simulink model "turbo_controller"  (R2025a)
settings: Solver=FixedStepAuto  StartTime=0.0  StopTime=inf  FixedStep=0.001  RelTol=1e-3
PostLoadFcn:
  | % 自动定位同目录CubeMX文件；不需要外部初始化脚本。
  | codertarget.data.setParameterValue('turbo_controller','STM32CubeMX.ProjectFile',fullfile(fileparts(get_param('turbo_controller','FileName')),'turbo_f407.ioc'));
InitFcn:
  | % 中文说明：按原控制器字段与类型创建三组接口总线；控制参数已内嵌。
  | tc_names=["EValve_Cycle" "EValve_Open" "Eblast_Cycle" "Eblast_Open" "Motor_Cycle" "Motor_Open" "EValve_Enable" "Eblast_Enable" "Motor_Enable" "SWO_Firework" "SWO_BleedAir" "EngineState" "Flag_ECUReset_Clear" "Flag_ECUReset_Save" "Flag_Reset_Enable" "Accelerator" "Nc_dem" "Nc"]; tc_types=["uint16" "uint16" "uint16" "uint16" "uint16" "uint16" "uint8" "uint8" "uint8" "uint8" "uint8" "uint8" "uint8" "uint8" "uint8" "single" "single" "single"];
  | for tc_k=1:numel(tc_names)
  |  tc_e(tc_k)=Simulink.BusElement; tc_e(tc_k).Name=char(tc_names(tc_k)); tc_e(tc_k).DataType=char(tc_types(tc_k));
  | end
  | EngineControl_Out=Simulink.Bus; EngineControl_Out.DataScope='Exported'; EngineControl_Out.Elements=tc_e;
  | clear tc_e tc_names tc_types tc_k
  | tc_names=["savedata1" "savedata2" "savedata3" "savedata4" "savedata5" "savedata6" "savedata7" "savedata8" "savedata9" "savedata10" "savedata11" "savedata12" "savedata13" "savedata14" "savedata15" "savedata16" "savedata17" "savedata18" "savedata19" "savedata20" "savedata21" "savedata22" "savedata23" "savedata24" "savedata25"]; tc_types=["single" "single" "single" "single" "single" "single" "single" "single" "single" "single" "single" "single" "single" "single" "single" "single" "single" "single" "single" "single" "single" "single" "single" "single" "single"];
  | for tc_k=1:numel(tc_names)
  |  tc_e(tc_k)=Simulink.BusElement; tc_e(tc_k).Name=char(tc_names(tc_k)); tc_e(tc_k).DataType=char(tc_types(tc_k));
  | end
  | SaveData_Out=Simulink.Bus; SaveData_Out.DataScope='Exported'; SaveData_Out.Elements=tc_e;
  | clear tc_e tc_names tc_types tc_k
  | tc_names=["senddata1" "senddata2" "senddata3" "senddata4" "senddata5" "senddata6" "senddata7" "senddata8" "senddata9" "senddata10" "senddata11" "senddata12" "senddata13" "senddata14" "senddata15" "senddata16" "senddata17" "senddata18" "senddata19" "senddata20" "senddata21" "senddata22" "senddata23" "senddata24" "senddata25" "senddata26" "senddata27" "senddata28" "senddata29"]; tc_types=["uint8" "uint8" "uint8" "uint8" "uint8" "uint8" "uint8" "uint8" "uint8" "uint8" "uint8" "uint8" "uint8" "uint8" "uint8" "uint8" "uint8" "uint8" "uint8" "uint8" "uint8" "uint8" "uint8" "uint8" "uint8" "uint8" "uint8" "uint8" "uint8"];
  | for tc_k=1:numel(tc_names)
  |  tc_e(tc_k)=Simulink.BusElement; tc_e(tc_k).Name=char(tc_names(tc_k)); tc_e(tc_k).DataType=char(tc_types(tc_k));
  | end
  | SendData_Out=Simulink.Bus; SendData_Out.DataScope='Exported'; SendData_Out.Elements=tc_e;
  | clear tc_e tc_names tc_types tc_k
  | 
  | % 以下为接口中文说明；只设置描述，不改变数值或数据类型。
  | EngineControl_Out.Description='执行控制输出（阀、电机、点火、状态及复位请求）';
  | tc_cn=["EValve_Cycle（主油阀周期计数（每计数2毫秒））" "EValve_Open（主油阀开通计数（每计数2毫秒））" "Eblast_Cycle（副油阀周期计数（每计数2毫秒））" "Eblast_Open（副油阀开通计数（每计数2毫秒））" "Motor_Cycle（起动电机周期计数）" "Motor_Open（起动电机开通计数）" "EValve_Enable（主油阀驱动使能）" "Eblast_Enable（副油阀驱动使能）" "Motor_Enable（起动电机使能）" "SWO_Firework（点火器使能（1开））" "SWO_BleedAir（引气阀使能（1开））" "EngineState（发动机状态）" "Flag_ECUReset_Clear（清除复位恢复状态请求）" "Flag_ECUReset_Save（保存复位恢复数据请求）" "Flag_Reset_Enable（处理器软件复位请求）" "Accelerator（油门／油泵给定控制量）" "Nc_dem（控制目标转速）" "Nc（发动机反馈转速（转每分））"];
  | tc_elements=EngineControl_Out.Elements;
  | for tc_k=1:numel(tc_cn)
  |  tc_elements(tc_k).Description=char(tc_cn(tc_k));
  | end
  | EngineControl_Out.Elements=tc_elements;
  | clear tc_cn tc_elements tc_k
  | SaveData_Out.Description='25项运行记录；字段含义按当前模型数据来源解释';
  | tc_cn=["savedata1（指令回显记录）" "savedata2（入口总温记录（℃））" "savedata3（电源电压记录）" "savedata4（排气温度记录（℃））" "savedata5（标定燃油压力记录）" "savedata6（副油阀占空比记录（％））" "savedata7（主油阀占空比记录（％））" "savedata8（温度修正转速记录）" "savedata9（开关输出及反馈位域）" "savedata10（物理转速记录）" "savedata11（油泵目标给定原始值）" "savedata12（起动电机占空比记录（％））" "savedata13（发动机状态码记录）" "savedata14（故障告警位域记录）" "savedata15（模型记录帧序号）" "savedata16（处理器温度记录（℃））" "savedata17（装订转速记录（沿用旧电源字段名））" "savedata18（导航高度记录）" "savedata19（飞行空速记录）" "savedata20（主阀旧记录位（恒零保留））" "savedata21（第21项保留记录（恒零））" "savedata22（保留记录项22）" "savedata23（保留记录项23）" "savedata24（保留记录项24）" "savedata25（保留记录项25）"];
  | tc_elements=SaveData_Out.Elements;
  | for tc_k=1:numel(tc_cn)
  |  tc_elements(tc_k).Description=char(tc_cn(tc_k));
  | end
  | SaveData_Out.Elements=tc_elements;
  | clear tc_cn tc_elements tc_k
  | SendData_Out.Description='29字段回传及外设命令接口；板端上位机帧只取第3至27字段';
  | tc_cn=["senddata1（回传发送允许标志（不直接上线路））" "senddata2（回传载荷长度25字节）" "senddata3（回传指令回显字节）" "senddata4（总温编码字节（℃＋80））" "senddata5（电源电压编码字节）" "senddata6（排温编码高字节）" "senddata7（排温编码低字节）" "senddata8（燃油压力编码高字节）" "senddata9（燃油压力编码低字节）" "senddata10（副油阀占空比字节（％））" "senddata11（主油阀占空比字节（％））" "senddata12（修正转速编码高字节）" "senddata13（修正转速编码低字节）" "senddata14（驱动及反馈状态位域）" "senddata15（物理转速编码高字节）" "senddata16（物理转速编码低字节）" "senddata17（油泵目标给定高字节（串口二使用））" "senddata18（油泵目标给定低字节（串口二使用））" "senddata19（起动电机占空比命令（串口一使用））" "senddata20（发动机状态码字节）" "senddata21（故障告警位域字节）" "senddata22（帧序号占位（板端另行填写））" "senddata23（处理器温度编码（℃＋50））" "senddata24（控制目标转速编码高字节）" "senddata25（控制目标转速编码低字节）" "senddata26（占位字节（板端改填实测泵速高字节））" "senddata27（占位字节（板端改填实测泵速低字节））" "senddata28（装订转速高字节（本板未发送））" "senddata29（装订转速低字节（本板未发送））"];
  | tc_elements=SendData_Out.Elements;
  | for tc_k=1:numel(tc_cn)
  |  tc_elements(tc_k).Description=char(tc_cn(tc_k));
  | end
  | SendData_Out.Elements=tc_elements;
  | clear tc_cn tc_elements tc_k
  | 
  | 
  | % FRAM模块化事务：接口类型和上电初始状态，随模型保存，无外部初始化文件。
  | clear FM_elements
  | FM_elements(1)=Simulink.BusElement;FM_elements(1).Name='phase';FM_elements(1).DataType='uint8';FM_elements(1).Dimensions=[1 1];FM_elements(1).Description='phase（当前事务阶段）';
  | FM_elements(2)=Simulink.BusElement;FM_elements(2).Name='a';FM_elements(2).DataType='uint8';FM_elements(2).Dimensions=[64 1];FM_elements(2).Description='a（启动时缓存的首区64字节）';
  | FM_elements(3)=Simulink.BusElement;FM_elements(3).Name='active';FM_elements(3).DataType='uint16';FM_elements(3).Dimensions=[1 1];FM_elements(3).Description='active（当前有效记录区地址）';
  | FM_elements(4)=Simulink.BusElement;FM_elements(4).Name='generation';FM_elements(4).DataType='uint32';FM_elements(4).Dimensions=[1 1];FM_elements(4).Description='generation（当前有效记录代号）';
  | FM_elements(5)=Simulink.BusElement;FM_elements(5).Name='record';FM_elements(5).DataType='uint8';FM_elements(5).Dimensions=[64 1];FM_elements(5).Description='record（本次冻结的待写记录）';
  | FM_elements(6)=Simulink.BusElement;FM_elements(6).Name='addr';FM_elements(6).DataType='uint16';FM_elements(6).Dimensions=[1 1];FM_elements(6).Description='addr（本次备用写入地址）';
  | FM_elements(7)=Simulink.BusElement;FM_elements(7).Name='lastSave';FM_elements(7).DataType='single';FM_elements(7).Dimensions=[1 1];FM_elements(7).Description='lastSave（上次开始保存的秒数）';
  | FM_elements(8)=Simulink.BusElement;FM_elements(8).Name='lastState';FM_elements(8).DataType='uint8';FM_elements(8).Dimensions=[1 1];FM_elements(8).Description='lastState（上次保存时的发动机状态）';
  | FM_elements(9)=Simulink.BusElement;FM_elements(9).Name='boot';FM_elements(9).DataType='boolean';FM_elements(9).Dimensions=[1 1];FM_elements(9).Description='boot（启动记录是否允许恢复）';
  | FM_elements(10)=Simulink.BusElement;FM_elements(10).Name='consumed';FM_elements(10).DataType='boolean';FM_elements(10).Dimensions=[1 1];FM_elements(10).Description='consumed（本次启动恢复通知是否已发送）';
  | FM_elements(11)=Simulink.BusElement;FM_elements(11).Name='payload';FM_elements(11).DataType='uint8';FM_elements(11).Dimensions=[20 1];FM_elements(11).Description='payload（当前20字节恢复内容）';
  | ... (+35 lines)
model workspace (MAT data in the model file):
  CRC16_Table_Reference = [0 4129 8258 12387 16516 20645 24774 28903 33032 37161 41290 45419 ... (256 elements, 256x1)]
  PE_Kaer = [0.15402 0.15402 0.12264 0.10076 0.09481 0.07601 0.07111 0.0569 0.05198 0.04926 0.05308 0.04325 ... (13 elements, 1x13)]
  PE_Nr = [21.2982 61.4260372 67.7475458 72.7394382 76.845934 80.6988798 83.8449282 86.6491912 88.9382406 89.178606 91.1938214 93.4068058 ... (13 elements, 1x13)]
  PE_Pump_Translate = 33.5999984741
  PE_RotaSpeed_Translate = 860
  PE_Taer = [0.4939154 0.4939154 0.40780982 0.34066978 0.31622756 0.30405716 0.34300244 0.26785022 0.37393554 0.23914836 0.44563948 0.31044662 ... (13 elements, 1x13)]
  PF_ACCFULLRANGE = 3360
  PF_Flag_ECUReset = 0
  PF_Flag_rx_suc = 1
  PF_Gear_Info = [40000; 45000; 50000; 55000; 57000; 59000; 60000; 61000; 61000; 61000; 61000; 61000]
  PF_K_TiaoJie = 1
  PF_Kpu = 10
  PF_MySet_Rxdata = [0 0 0 0 0 0 0 0 0 0 0 0 ... (50 elements, 50x1)]
  PF_MyUsart1_Rxdata = [0 0 0 0 0 0 0 0 0 0 0 0 ... (50 elements, 50x1)]
  PF_MyUsart2_Rxdata = [0 0 0 0 0 0 0 0 0 0 0 0 ... (50 elements, 50x1)]
  PF_Reset_Information = [0 0 0 0 0 0 0 0 0 0 0 0 ... (20 elements, 20x1)]
  PF_Sensor_X1_T4 = [0 4095]
  PF_Sensor_X2_T4 = [0 1.66666698456]
  PF_Sensor_X3_T4 = [0 504 999 1497 2010 2529 3051 3568 4076 4571 4959]
  PF_Sensor_X_P2 = [0.5 3]
  PF_Sensor_X_Poil = [0.5 3]
  PF_Sensor_X_T1t = [-50 300]
  PF_Sensor_X_Vpower = [0 3]
  PF_Sensor_X_Vpump = [0 3]
  PF_Sensor_Y1_T4 = [0 3]
  PF_Sensor_Y2_T4 = [0 5000]
  PF_Sensor_Y3_T4 = [0 100 200 300 400 500 600 700 800 900 980]
  PF_Sensor_Y_P2 = [0 1000]
  PF_Sensor_Y_Poil = [0 1000]
  PF_Sensor_Y_T1t = [-50 300]
  PF_Sensor_Y_Vpower = [0 33]
  PF_Sensor_Y_Vpump = [0 33]
  PG_CtrlMode_CloseLoop : mpt.Parameter (value not decoded)
  PG_CtrlMode_ManualAcc : mpt.Parameter (value not decoded)
  PG_CtrlMode_Origin : mpt.Parameter (value not decoded)
  PG_CtrlMode_Start : mpt.Parameter (value not decoded)
  PG_CtrlMode_Stop : mpt.Parameter (value not decoded)
  PG_ES_Clp : mpt.Parameter (value not decoded)
  PG_ES_EngStart : mpt.Parameter (value not decoded)
  PG_ES_Manual : mpt.Parameter (value not decoded)
  PG_ES_Origin : mpt.Parameter (value not decoded)
  PG_ES_Stop : mpt.Parameter (value not decoded)
  PG_Instr_BleedAirSet : mpt.Parameter (value not decoded)
  PG_Instr_CloseLoop : mpt.Parameter (value not decoded)
  PG_Instr_ECUReSet : mpt.Parameter (value not decoded)
  PG_Instr_EValveSet : mpt.Parameter (value not decoded)
  PG_Instr_EblastSet : mpt.Parameter (value not decoded)
  PG_Instr_Erase : mpt.Parameter (value not decoded)
  PG_Instr_FireWorkSet : mpt.Parameter (value not decoded)
  PG_Instr_ManualPlus : mpt.Parameter (value not decoded)
  PG_Instr_ManualrReduce : mpt.Parameter (value not decoded)
  PG_Instr_MotorSet : mpt.Parameter (value not decoded)
  PG_Instr_OilSet : mpt.Parameter (value not decoded)
  PG_Instr_SelfCheck : mpt.Parameter (value not decoded)
  PG_Instr_Start : mpt.Parameter (value not decoded)
  PG_Instr_Stop : mpt.Parameter (value not decoded)
  PG_Instr_StopZero : Simulink.Parameter (value not decoded)
  PG_Location_Air : Simulink.Parameter (value not decoded)
  PG_Location_Gnd : Simulink.Parameter (value not decoded)
  PG_ServoCtrlMode_CloseLoop : Simulink.Parameter (value not decoded)
  PG_ServoCtrlMode_CloseLoopMax : Simulink.Parameter (value not decoded)
  PG_ServoCtrlMode_CloseLoopMin : Simulink.Parameter (value not decoded)
  PG_ServoCtrlMode_ManualAcc : Simulink.Parameter (value not decoded)
  PG_ServoCtrlMode_ManualAccMax : Simulink.Parameter (value not decoded)
  PG_ServoCtrlMode_ManualAccMin : Simulink.Parameter (value not decoded)
  PG_SpeedDot_Permit : Simulink.Parameter (value not decoded)
  PL_EngineModel_Actuator = [0 10 100]
  PL_EngineModel_EngineStar_Press_P2 = [1013 1098.4 1099.144828 1099.931034 1103.613793 1162.662069 1143.793103 1131.006897 1123.186207 1117.6 1114 1111.806897 ... (127 elements, 1x127)]
  PL_EngineModel_EngineStar_RotaSpeed = [200 2000 9584 9660 10220 10240 10260 10288 10308 10368 10380 10408 ... (127 elements, 1x127)]
  PL_EngineModel_EngineStar_Temp_Exhaust = [128 129 129.1 130 131 131.1 132 133 134 134.1 135 135.1 ... (127 elements, 1x127)]
  PL_EngineModel_EngineStar_Time = [0.05 0.1 0.15 0.2 0.25 0.3 0.35 0.4 0.45 0.5 0.55 0.6 ... (127 elements, 1x127)]
  PL_EngineModel_IdleAbove_Nr = [0 21.2982 61.4260372 67.7475458 72.7394382 76.845934 80.6988798 83.8449282 86.6491912 88.9382406 89.178606 91.1938214 ... (14 elements, 1x14)]
  PL_EngineModel_IdleAbove_P2r = [0.986923266716 1.57907722675 1.81593881076 1.99358499877 2.23044658278 2.43770046879 2.65482358747 2.84233900814 3.03972366149 3.18776215149 3.25684678016 3.3950160375 ... (14 elements, 1x14)]
  PL_EngineModel_IdleAbove_Tempr = [0.0536001429337 1.07200285867 1.63301768805 1.63659103091 1.66875111667 1.72592460247 1.77595140254 1.86171163123 1.95461854565 2.03323208862 2.03323208862 2.13685903162 ... (14 elements, 1x14)]
  PL_EngineModel_IdleAbove_Ter = [0.42434128 0.42434128 0.42434128 0.30669408 0.23570008 0.22150128 0.1997974 0.23803274 0.16115638 0.24279948 0.13600422 0.31308354 ... (14 elements, 1x14)]
  PL_EngineModel_IdleAbove_Wfr = [0 10.142 23.8337 27.8905 31.9473 36.0041 40.0609 44.1177 48.1745 52.2313 52.7384 56.7952 ... (14 elements, 1x14)]
  PL_EngineModel_Press_P2 = [400 400 400 400 400 400 400 400 400 400]
  PL_EngineModel_Rotaspeed = [0 20000 96400]
  PL_EngineModel_Temp_Exhaust = [500 500 500 500 500 500 500 500 500 500]
  PL_Kaer = [0.1 0.1 0.1 0.1 0.1 0.1]
  PL_Nr = [50 60 70 80 90 100]
  PL_Taer = [0.1 0.1 0.1 0.1 0.1 0.1]
  Sig : Simulink.Signal (value not decoded)
  Ts_ms : Simulink.Parameter (value not decoded)
  false : Simulink.Parameter (value not decoded)
  true : Simulink.Parameter (value not decoded)
symbols that are objects in the model workspace (value not decoded): PG_CtrlMode_CloseLoop, PG_CtrlMode_ManualAcc, PG_CtrlMode_Origin, PG_CtrlMode_Start, PG_CtrlMode_Stop, PG_ES_Clp, PG_ES_EngStart, PG_ES_Manual, PG_ES_Origin, PG_ES_Stop, PG_Instr_BleedAirSet, PG_Instr_CloseLoop, PG_Instr_EblastSet, PG_Instr_ECUReSet, PG_Instr_Erase, PG_Instr_EValveSet, PG_Instr_FireWorkSet, PG_Instr_ManualPlus, PG_Instr_ManualrReduce, PG_Instr_MotorSet, PG_Instr_OilSet, PG_Instr_SelfCheck, PG_Instr_Start, PG_Instr_Stop, PG_Instr_StopZero, PG_ServoCtrlMode_CloseLoop, PG_ServoCtrlMode_CloseLoopMax, PG_ServoCtrlMode_CloseLoopMin, PG_ServoCtrlMode_ManualAcc, PG_ServoCtrlMode_ManualAccMax, PG_ServoCtrlMode_ManualAccMin, Ts_ms
libraries: simulink x97, stm32blockslib x10, stm32f4xxblockslib x8
(part 15 of 26)

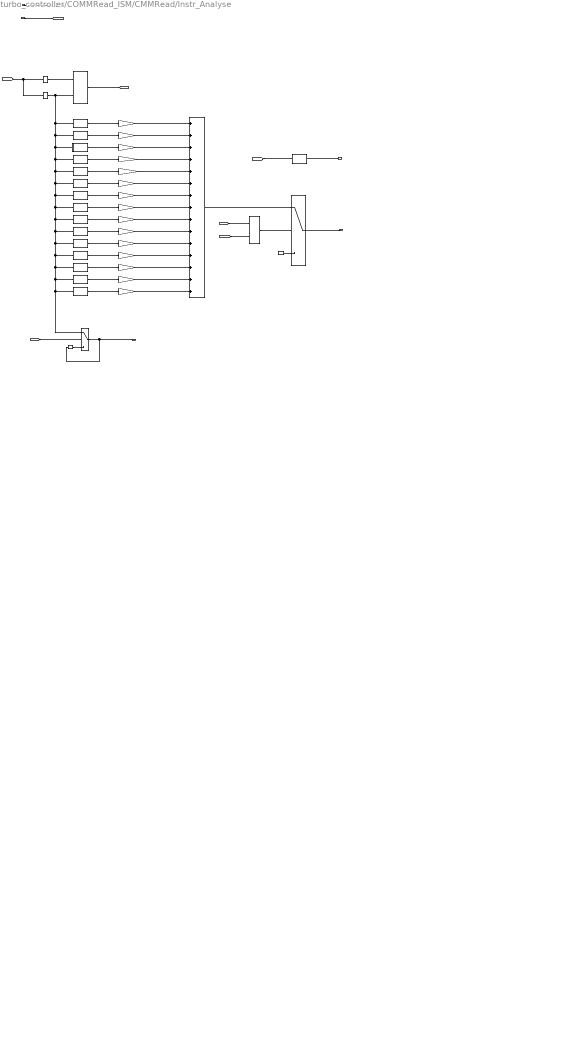
== system turbo_controller/COMMRead_ISM/CMMRead/Instr_Analyse ==
  note: 指令分析模型（仅针对触发式通信方式）：
      | 按照P40WP_B的通信协议给出。
      | 不具备连续计算空中状态 的能力。
  note: 【本页库子系统中文说明】ShouDongJia
      | 一、它做什么？
      | 这是“过不过这条线”的判断器。将输入与阈值 uint8(hex2dec('F1')) 作 == 比较，
      | 关系成立输出真（1），否则输出假（0）。例如>=包含恰好等于，>则不包含。它只给
      | 出判断标志，不会自行限幅、报警、切换状态或操作阀门；后续逻辑决定如何使用。名
      | 称可能只是用途提示，实际判据以这里的关系和阈值为准。
      | 二、本实例当前参数
      | 比较关系：==
      | 比较阈值：uint8(hex2dec('F1'))
      | 输出数据类型：uint8
      | 零交叉检测：开启
      | 三、怎样继续学习？
      | 这是标准库子系统实例。中文说明放在使用它的父级页面，并同步存入本块Descriptio
      | n（模块说明）；官方库链接保留。先看本实例的输入来自哪里、输出交给谁，再结合
      | 以上参数理解作用。
  note: 【本页库子系统中文说明】cachu
      | 一、它做什么？
      | 这是“过不过这条线”的判断器。将输入与阈值 uint8(hex2dec('E4')) 作 == 比较，
      | 关系成立输出真（1），否则输出假（0）。例如>=包含恰好等于，>则不包含。它只给
      | 出判断标志，不会自行限幅、报警、切换状态或操作阀门；后续逻辑决定如何使用。名
      | 称可能只是用途提示，实际判据以这里的关系和阈值为准。
      | 二、本实例当前参数
      | 比较关系：==
      | 比较阈值：uint8(hex2dec('E4'))
      | 输出数据类型：uint8
      | 零交叉检测：开启
      | 三、怎样继续学习？
      | 这是标准库子系统实例。中文说明放在使用它的父级页面，并同步存入本块Descriptio
      | n（模块说明）；官方库链接保留。先看本实例的输入来自哪里、输出交给谁，再结合
      | 以上参数理解作用。
  note: 【本页库子系统中文说明】chongzhi
      | 一、它做什么？
      | 这是“过不过这条线”的判断器。将输入与阈值 uint8(hex2dec('F4')) 作 == 比较，
      | 关系成立输出真（1），否则输出假（0）。例如>=包含恰好等于，>则不包含。它只给
      | 出判断标志，不会自行限幅、报警、切换状态或操作阀门；后续逻辑决定如何使用。名
      | 称可能只是用途提示，实际判据以这里的关系和阈值为准。
      | 二、本实例当前参数
      | 比较关系：==
      | 比较阈值：uint8(hex2dec('F4'))
      | 输出数据类型：uint8
      | 零交叉检测：开启
      | 三、怎样继续学习？
      | 这是标准库子系统实例。中文说明放在使用它的父级页面，并同步存入本块Descriptio
      | n（模块说明）；官方库链接保留。先看本实例的输入来自哪里、输出交给谁，再结合
      | 以上参数理解作用。
  note: 【本页库子系统中文说明】jinjitingche
      | 一、它做什么？
      | 这是“过不过这条线”的判断器。将输入与阈值 uint8(hex2dec('A1')) 作 == 比较，
      | 关系成立输出真（1），否则输出假（0）。例如>=包含恰好等于，>则不包含。它只给
      | 出判断标志，不会自行限幅、报警、切换状态或操作阀门；后续逻辑决定如何使用。名
      | 称可能只是用途提示，实际判据以这里的关系和阈值为准。
      | 二、本实例当前参数
      | 比较关系：==
      | 比较阈值：uint8(hex2dec('A1'))
      | 输出数据类型：uint8
      | 零交叉检测：开启
      | 三、怎样继续学习？
      | 这是标准库子系统实例。中文说明放在使用它的父级页面，并同步存入本块Descriptio
      | n（模块说明）；官方库链接保留。先看本实例的输入来自哪里、输出交给谁，再结合
      | 以上参数理解作用。
  note: 【本页库子系统中文说明】qidong
      | 一、它做什么？
      | 这是“过不过这条线”的判断器。将输入与阈值 uint8(hex2dec('FC')) 作 == 比较，
      | 关系成立输出真（1），否则输出假（0）。例如>=包含恰好等于，>则不包含。它只给
      | 出判断标志，不会自行限幅、报警、切换状态或操作阀门；后续逻辑决定如何使用。名
      | 称可能只是用途提示，实际判据以这里的关系和阈值为准。
      | 二、本实例当前参数
      | 比较关系：==
      | 比较阈值：uint8(hex2dec('FC'))
      | 输出数据类型：uint8
      | 零交叉检测：开启
      | 三、怎样继续学习？
      | 这是标准库子系统实例。中文说明放在使用它的父级页面，并同步存入本块Descriptio
      | n（模块说明）；官方库链接保留。先看本实例的输入来自哪里、输出交给谁，再结合
      | 以上参数理解作用。
  note: 【本页库子系统中文说明】shedingDianHuoQi
      | 一、它做什么？
      | 这是“过不过这条线”的判断器。将输入与阈值 uint8(hex2dec('E2')) 作 == 比较，
      | 关系成立输出真（1），否则输出假（0）。例如>=包含恰好等于，>则不包含。它只给
      | 出判断标志，不会自行限幅、报警、切换状态或操作阀门；后续逻辑决定如何使用。名
      | 称可能只是用途提示，实际判据以这里的关系和阈值为准。
      | 二、本实例当前参数
      | 比较关系：==
      | 比较阈值：uint8(hex2dec('E2'))
      | 输出数据类型：uint8
      | 零交叉检测：开启
      | 三、怎样继续学习？
      | 这是标准库子系统实例。中文说明放在使用它的父级页面，并同步存入本块Descriptio
      | n（模块说明）；官方库链接保留。先看本实例的输入来自哪里、输出交给谁，再结合
      | 以上参数理解作用。
  note: 【本页库子系统中文说明】shedingDianJi
      | 一、它做什么？
      | 这是“过不过这条线”的判断器。将输入与阈值 uint8(hex2dec('E8')) 作 == 比较，
      | 关系成立输出真（1），否则输出假（0）。例如>=包含恰好等于，>则不包含。它只给
      | 出判断标志，不会自行限幅、报警、切换状态或操作阀门；后续逻辑决定如何使用。名
      | 称可能只是用途提示，实际判据以这里的关系和阈值为准。
      | 二、本实例当前参数
      | 比较关系：==
      | 比较阈值：uint8(hex2dec('E8'))
      | 输出数据类型：uint8
      | 零交叉检测：开启
      | 三、怎样继续学习？
      | 这是标准库子系统实例。中文说明放在使用它的父级页面，并同步存入本块Descriptio
      | n（模块说明）；官方库链接保留。先看本实例的输入来自哪里、输出交给谁，再结合
      | 以上参数理解作用。
  note: 【本页库子系统中文说明】shedingFuFa
      | 一、它做什么？
      | 这是“过不过这条线”的判断器。将输入与阈值 uint8(hex2dec('E7')) 作 == 比较，
      | 关系成立输出真（1），否则输出假（0）。例如>=包含恰好等于，>则不包含。它只给
      | 出判断标志，不会自行限幅、报警、切换状态或操作阀门；后续逻辑决定如何使用。名
      | 称可能只是用途提示，实际判据以这里的关系和阈值为准。
      | 二、本实例当前参数
      | 比较关系：==
      | 比较阈值：uint8(hex2dec('E7'))
      | 输出数据类型：uint8
      | 零交叉检测：开启
      | 三、怎样继续学习？
      | 这是标准库子系统实例。中文说明放在使用它的父级页面，并同步存入本块Descriptio
      | n（模块说明）；官方库链接保留。先看本实例的输入来自哪里、输出交给谁，再结合
      | 以上参数理解作用。
  note: 【本页库子系统中文说明】shedingZhuFa
      | 一、它做什么？
      | 这是“过不过这条线”的判断器。将输入与阈值 uint8(hex2dec('E6')) 作 == 比较，
      | 关系成立输出真（1），否则输出假（0）。例如>=包含恰好等于，>则不包含。它只给
      | 出判断标志，不会自行限幅、报警、切换状态或操作阀门；后续逻辑决定如何使用。名
      | 称可能只是用途提示，实际判据以这里的关系和阈值为准。
      | 二、本实例当前参数
      | 比较关系：==
      | 比较阈值：uint8(hex2dec('E6'))
      | 输出数据类型：uint8
      | 零交叉检测：开启
      | 三、怎样继续学习？
      | 这是标准库子系统实例。中文说明放在使用它的父级页面，并同步存入本块Descriptio
      | n（模块说明）；官方库链接保留。先看本实例的输入来自哪里、输出交给谁，再结合
      | 以上参数理解作用。
  note: 【本页库子系统中文说明】shedingyingqi
      | 一、它做什么？
      | 这是“过不过这条线”的判断器。将输入与阈值 uint8(hex2dec('E9')) 作 == 比较，
      | 关系成立输出真（1），否则输出假（0）。例如>=包含恰好等于，>则不包含。它只给
      | 出判断标志，不会自行限幅、报警、切换状态或操作阀门；后续逻辑决定如何使用。名
      | 称可能只是用途提示，实际判据以这里的关系和阈值为准。
      | 二、本实例当前参数
      | 比较关系：==
      | 比较阈值：uint8(hex2dec('E9'))
      | 输出数据类型：uint8
      | 零交叉检测：开启
      | 三、怎样继续学习？
      | 这是标准库子系统实例。中文说明放在使用它的父级页面，并同步存入本块Descriptio
      | n（模块说明）；官方库链接保留。先看本实例的输入来自哪里、输出交给谁，再结合
      | 以上参数理解作用。
  note: 【本页库子系统中文说明】shedingyoumen
      | 一、它做什么？
      | 这是“过不过这条线”的判断器。将输入与阈值 uint8(hex2dec('E3')) 作 == 比较，
      | 关系成立输出真（1），否则输出假（0）。例如>=包含恰好等于，>则不包含。它只给
      | 出判断标志，不会自行限幅、报警、切换状态或操作阀门；后续逻辑决定如何使用。名
      | 称可能只是用途提示，实际判据以这里的关系和阈值为准。
      | 二、本实例当前参数
      | 比较关系：==
      | 比较阈值：uint8(hex2dec('E3'))
      | 输出数据类型：uint8
      | 零交叉检测：开启
      | 三、怎样继续学习？
      | 这是标准库子系统实例。中文说明放在使用它的父级页面，并同步存入本块Descriptio
      | n（模块说明）；官方库链接保留。先看本实例的输入来自哪里、输出交给谁，再结合
      | 以上参数理解作用。
  note: 【本页库子系统中文说明】shoudongjian
      | 一、它做什么？
      | 这是“过不过这条线”的判断器。将输入与阈值 uint8(hex2dec('F2')) 作 == 比较，
      | 关系成立输出真（1），否则输出假（0）。例如>=包含恰好等于，>则不包含。它只给
      | 出判断标志，不会自行限幅、报警、切换状态或操作阀门；后续逻辑决定如何使用。名
      | 称可能只是用途提示，实际判据以这里的关系和阈值为准。
      | 二、本实例当前参数
      | 比较关系：==
      | 比较阈值：uint8(hex2dec('F2'))
      | 输出数据类型：uint8
      | 零交叉检测：开启
      | 三、怎样继续学习？
      | 这是标准库子系统实例。中文说明放在使用它的父级页面，并同步存入本块Descriptio
      | n（模块说明）；官方库链接保留。先看本实例的输入来自哪里、输出交给谁，再结合
      | 以上参数理解作用。
  note: 【本页库子系统中文说明】tingche
      | 一、它做什么？
      | 这是“过不过这条线”的判断器。将输入与阈值 uint8(hex2dec('F0')) 作 == 比较，
      | 关系成立输出真（1），否则输出假（0）。例如>=包含恰好等于，>则不包含。它只给
      | 出判断标志，不会自行限幅、报警、切换状态或操作阀门；后续逻辑决定如何使用。名
      | 称可能只是用途提示，实际判据以这里的关系和阈值为准。
      | 二、本实例当前参数
      | 比较关系：==
      | 比较阈值：uint8(hex2dec('F0'))
      | 输出数据类型：uint8
      | 零交叉检测：开启
      | 三、怎样继续学习？
      | 这是标准库子系统实例。中文说明放在使用它的父级页面，并同步存入本块Descriptio
      | n（模块说明）；官方库链接保留。先看本实例的输入来自哪里、输出交给谁，再结合
      | 以上参数理解作用。
  note: 【本页库子系统中文说明】zijian
      | 一、它做什么？
      | 这是“过不过这条线”的判断器。将输入与阈值 uint8(hex2dec('E1')) 作 == 比较，
      | 关系成立输出真（1），否则输出假（0）。例如>=包含恰好等于，>则不包含。它只给
      | 出判断标志，不会自行限幅、报警、切换状态或操作阀门；后续逻辑决定如何使用。名
      | 称可能只是用途提示，实际判据以这里的关系和阈值为准。
      | 二、本实例当前参数
      | 比较关系：==
      | 比较阈值：uint8(hex2dec('E1'))
      | 输出数据类型：uint8
      | 零交叉检测：开启
      | 三、怎样继续学习？
      | 这是标准库子系统实例。中文说明放在使用它的父级页面，并同步存入本块Descriptio
      | n（模块说明）；官方库链接保留。先看本实例的输入来自哪里、输出交给谁，再结合
      | 以上参数理解作用。
  note: 识别上位机命令，并把相关数据交给对应功能
      |
      | 从已接收帧中取出命令字段，将其与起动、停车、闭环、手动泵、阀门、电机、点火及引气等命令常量
      | 比较。带有效接收条件的选择支路更新本次指令和参数，否则保持原先设定。
      |
      | 装订/档位另有复合编码识别，不是把整个命令字直接当作一个状态编号。输出同时包含指令结果、成
      | 功标志和需要继续解释的数据。
      |
      | 指令描述“用户要求做什么”，EngineState描述“发动机当前处于什么模式”，两者不是一个变量。
      | 指令先进入ESM产生模式转换条件，再由CLM选择控制分支；不能因收到一条Start就认为硬件已经起动
      | 完成。
  note: ShouDongJia
      | ShouDongJia：只判断一个条件
      |
      | 把输入与0xF1（十进制241）比较，使用关系“==”。成立输出1，不成立输出0；输出是判断标志，不
      | 是把输入缩放成该常数。
      |
      | 这里识别一种指令编码。判断成立只说明指令匹配；父级还会结合有效帧、当前模式或其他允许条件决
      | 定是否更新。实际驱动要继续经过控制与板级输出，不能把1理解为硬件执行回执。
  note: cachu
      | cachu：只判断一个条件
      |
      | 把输入与0xE4（十进制228）比较，使用关系“==”。成立输出1，不成立输出0；输出是判断标志，不
      | 是把输入缩放成该常数。
      |
      | 这里识别一种指令编码。判断成立只说明指令匹配；父级还会结合有效帧、当前模式或其他允许条件决
      | 定是否更新。实际驱动要继续经过控制与板级输出，不能把1理解为硬件执行回执。
  note: chongzhi
      | chongzhi：只判断一个条件
      |
      | 把输入与0xF4（十进制244）比较，使用关系“==”。成立输出1，不成立输出0；输出是判断标志，不
      | 是把输入缩放成该常数。
      |
      | 这里识别一种指令编码。判断成立只说明指令匹配；父级还会结合有效帧、当前模式或其他允许条件决
      | 定是否更新。实际驱动要继续经过控制与板级输出，不能把1理解为硬件执行回执。
  note: jinjitingche
      | jinjitingche：只判断一个条件
      |
      | 把输入与0xA1（十进制161）比较，使用关系“==”。成立输出1，不成立输出0；输出是判断标志，不
      | 是把输入缩放成该常数。
      |
      | 这里识别一种指令编码。判断成立只说明指令匹配；父级还会结合有效帧、当前模式或其他允许条件决
      | 定是否更新。实际驱动要继续经过控制与板级输出，不能把1理解为硬件执行回执。
  note: qidong
      | qidong：只判断一个条件
      |
      | 把输入与0xFC（十进制252）比较，使用关系“==”。成立输出1，不成立输出0；输出是判断标志，不
      | 是把输入缩放成该常数。
      |
      | 这里识别一种指令编码。判断成立只说明指令匹配；父级还会结合有效帧、当前模式或其他允许条件决
      | 定是否更新。实际驱动要继续经过控制与板级输出，不能把1理解为硬件执行回执。
  note: shedingDianHuoQi
      | shedingDianHuoQi：只判断一个条件
      |
      | 把输入与0xE2（十进制226）比较，使用关系“==”。成立输出1，不成立输出0；输出是判断标志，不
      | 是把输入缩放成该常数。
      |
      | 这里识别一种指令编码。判断成立只说明指令匹配；父级还会结合有效帧、当前模式或其他允许条件决
      | 定是否更新。实际驱动要继续经过控制与板级输出，不能把1理解为硬件执行回执。
  note: shedingDianJi
      | shedingDianJi：只判断一个条件
      |
      | 把输入与0xE8（十进制232）比较，使用关系“==”。成立输出1，不成立输出0；输出是判断标志，不
      | 是把输入缩放成该常数。
      |
      | 这里识别一种指令编码。判断成立只说明指令匹配；父级还会结合有效帧、当前模式或其他允许条件决
      | 定是否更新。实际驱动要继续经过控制与板级输出，不能把1理解为硬件执行回执。
  note: shedingFuFa
      | shedingFuFa：只判断一个条件
      |
      | 把输入与0xE7（十进制231）比较，使用关系“==”。成立输出1，不成立输出0；输出是判断标志，不
      | 是把输入缩放成该常数。
      |
      | 这里识别一种指令编码。判断成立只说明指令匹配；父级还会结合有效帧、当前模式或其他允许条件决
      | 定是否更新。实际驱动要继续经过控制与板级输出，不能把1理解为硬件执行回执。
  note: shedingZhuFa
      | shedingZhuFa：只判断一个条件
      |
      | 把输入与0xE6（十进制230）比较，使用关系“==”。成立输出1，不成立输出0；输出是判断标志，不
      | 是把输入缩放成该常数。
      |
      | 这里识别一种指令编码。判断成立只说明指令匹配；父级还会结合有效帧、当前模式或其他允许条件决
      | 定是否更新。实际驱动要继续经过控制与板级输出，不能把1理解为硬件执行回执。
  note: shedingyingqi
      | shedingyingqi：只判断一个条件
      |
      | 把输入与0xE9（十进制233）比较，使用关系“==”。成立输出1，不成立输出0；输出是判断标志，不
      | 是把输入缩放成该常数。
      |
      | 这里识别一种指令编码。判断成立只说明指令匹配；父级还会结合有效帧、当前模式或其他允许条件决
      | 定是否更新。实际驱动要继续经过控制与板级输出，不能把1理解为硬件执行回执。
  note: shedingyoumen
      | shedingyoumen：只判断一个条件
      |
      | 把输入与0xE3（十进制227）比较，使用关系“==”。成立输出1，不成立输出0；输出是判断标志，不
      | 是把输入缩放成该常数。
      |
      | 这里识别一种指令编码。判断成立只说明指令匹配；父级还会结合有效帧、当前模式或其他允许条件决
      | 定是否更新。实际驱动要继续经过控制与板级输出，不能把1理解为硬件执行回执。
  note: shoudongjian
      | shoudongjian：只判断一个条件
      |
      | 把输入与0xF2（十进制242）比较，使用关系“==”。成立输出1，不成立输出0；输出是判断标志，不
      | 是把输入缩放成该常数。
      |
      | 这里识别一种指令编码。判断成立只说明指令匹配；父级还会结合有效帧、当前模式或其他允许条件决
      | 定是否更新。实际驱动要继续经过控制与板级输出，不能把1理解为硬件执行回执。
  note: tingche
      | tingche：只判断一个条件
      |
      | 把输入与0xF0（十进制240）比较，使用关系“==”。成立输出1，不成立输出0；输出是判断标志，不
      | 是把输入缩放成该常数。
      |
      | 这里识别一种指令编码。判断成立只说明指令匹配；父级还会结合有效帧、当前模式或其他允许条件决
      | 定是否更新。实际驱动要继续经过控制与板级输出，不能把1理解为硬件执行回执。
  note: zijian
      | zijian：只判断一个条件
      |
      | 把输入与0xE1（十进制225）比较，使用关系“==”。成立输出1，不成立输出0；输出是判断标志，不
      | 是把输入缩放成该常数。
      |
      | 这里识别一种指令编码。判断成立只说明指令匹配；父级还会结合有效帧、当前模式或其他允许条件决
      | 定是否更新。实际驱动要继续经过控制与板级输出，不能把1理解为硬件执行回执。
  S_MyUsart2_Rxdata : Inport
      settings: AttributesFormatString=S_MyUsart2_Rxdata（四号串口指令缓冲区（沿用旧变量名））
  S_Rx_suc : Inport  Port=2
      settings: AttributesFormatString=S_Rx_suc（接收数据成功或有效）
  Add : Sum  Inputs=15  OutDataTypeStr=uint8
      settings: AttributesFormatString=Add（加法求和）
  COMM数组3位 : Selector  IndexMode=Zero-based  InputPortWidth=50  IndexOptions=Index vector (dialog)  Indices=[2]  OutputSizes=1
      settings: AttributesFormatString=COMM数组3位（通信数组3位）
  COMM数组4位 : Selector  IndexMode=Zero-based  InputPortWidth=50  IndexOptions=Index vector (dialog)  Indices=[3]  OutputSizes=1
      settings: AttributesFormatString=COMM数组4位（通信数组4位）
  COMM数组6位 : Selector  IndexMode=Zero-based  InputPortWidth=50  IndexOptions=Index vector (dialog)  Indices=[5]  OutputSizes=1
      settings: AttributesFormatString=COMM数组6位（通信数组6位）
  Delay : Delay  DelayLength=1  InitialCondition=0
      settings: AttributesFormatString=Delay（延迟）
  ECU重置 : Gain  Gain=PG_Instr_ECUReSet
      settings: AttributesFormatString=ECU重置（控制器重置）
  ShouDongJia : simulink/Logic and Bit Operations/Compare To Constant  Description=|  relop===  const=uint8(hex2dec('F1'))  OutDataTypeStr=uint8
      | ShouDongJia：只判断一个条件
      | 
      | 把输入与0xF1（十进制241）比较，使用关系“==”。成立输出1，不成立输出0；输出是判断标志，不是把输入缩放成该常数。
      | 
      | 这里识别一种指令编码。判断成立只说明指令匹配；父级还会结合有效帧、当前模式或其他允许条件决定是否更新。实际驱动要继续经过控制与板级输出，不能把1理解为硬件执行回执。
      settings: AttributesFormatString=ShouDongJia（手动增加）
  Switch : Switch  Criteria=u2 ~= 0  SaturateOnIntegerOverflow=off  InputSameDT=off
      settings: AttributesFormatString=Switch（开关选择）
  Switch1 : Switch  Criteria=u2 ~= 0  SaturateOnIntegerOverflow=off  InputSameDT=off
      settings: AttributesFormatString=Switch（开关选择）
  WuZhiLing : Constant  Value=0  OutDataTypeStr=uint8
      settings: AttributesFormatString=WuZhiLing（无指令）
  cachu : simulink/Logic and Bit Operations/Compare To Constant  Description=|  relop===  const=uint8(hex2dec('E4'))  OutDataTypeStr=uint8
      | cachu：只判断一个条件
      | 
      | 把输入与0xE4（十进制228）比较，使用关系“==”。成立输出1，不成立输出0；输出是判断标志，不是把输入缩放成该常数。
      | 
      | 这里识别一种指令编码。判断成立只说明指令匹配；父级还会结合有效帧、当前模式或其他允许条件决定是否更新。实际驱动要继续经过控制与板级输出，不能把1理解为硬件执行回执。
      settings: AttributesFormatString=cachu（擦除）
  chongzhi : simulink/Logic and Bit Operations/Compare To Constant  Description=|  relop===  const=uint8(hex2dec('F4'))  OutDataTypeStr=uint8
      | chongzhi：只判断一个条件
      | 
      | 把输入与0xF4（十进制244）比较，使用关系“==”。成立输出1，不成立输出0；输出是判断标志，不是把输入缩放成该常数。
      | 
      | 这里识别一种指令编码。判断成立只说明指令匹配；父级还会结合有效帧、当前模式或其他允许条件决定是否更新。实际驱动要继续经过控制与板级输出，不能把1理解为硬件执行回执。
      settings: AttributesFormatString=chongzhi（重置）
  jinjitingche : simulink/Logic and Bit Operations/Compare To Constant  Description=|  relop===  const=uint8(hex2dec('A1'))  OutDataTypeStr=uint8
      | jinjitingche：只判断一个条件
      | 
      | 把输入与0xA1（十进制161）比较，使用关系“==”。成立输出1，不成立输出0；输出是判断标志，不是把输入缩放成该常数。
      | 
      | 这里识别一种指令编码。判断成立只说明指令匹配；父级还会结合有效帧、当前模式或其他允许条件决定是否更新。实际驱动要继续经过控制与板级输出，不能把1理解为硬件执行回执。
      settings: AttributesFormatString=jinjitingche（紧急停车）
  qidong : simulink/Logic and Bit Operations/Compare To Constant  Description=|  relop===  const=uint8(hex2dec('FC'))  OutDataTypeStr=uint8
      | qidong：只判断一个条件
      | 
      | 把输入与0xFC（十进制252）比较，使用关系“==”。成立输出1，不成立输出0；输出是判断标志，不是把输入缩放成该常数。
      | 
      | 这里识别一种指令编码。判断成立只说明指令匹配；父级还会结合有效帧、当前模式或其他允许条件决定是否更新。实际驱动要继续经过控制与板级输出，不能把1理解为硬件执行回执。
      settings: AttributesFormatString=qidong（起动）
  shedingDianHuoQi : simulink/Logic and Bit Operations/Compare To Constant  Description=|  relop===  const=uint8(hex2dec('E2'))  OutDataTypeStr=uint8
      | shedingDianHuoQi：只判断一个条件
      | 
      | 把输入与0xE2（十进制226）比较，使用关系“==”。成立输出1，不成立输出0；输出是判断标志，不是把输入缩放成该常数。
      | 
      | 这里识别一种指令编码。判断成立只说明指令匹配；父级还会结合有效帧、当前模式或其他允许条件决定是否更新。实际驱动要继续经过控制与板级输出，不能把1理解为硬件执行回执。
      settings: AttributesFormatString=shedingDianHuoQi（设定点火器）
  shedingDianJi : simulink/Logic and Bit Operations/Compare To Constant  Description=|  relop===  const=uint8(hex2dec('E8'))  OutDataTypeStr=uint8
      | shedingDianJi：只判断一个条件
      | 
      | 把输入与0xE8（十进制232）比较，使用关系“==”。成立输出1，不成立输出0；输出是判断标志，不是把输入缩放成该常数。
      | 
      | 这里识别一种指令编码。判断成立只说明指令匹配；父级还会结合有效帧、当前模式或其他允许条件决定是否更新。实际驱动要继续经过控制与板级输出，不能把1理解为硬件执行回执。
      settings: AttributesFormatString=shedingDianJi（设定电机）
  shedingFuFa : simulink/Logic and Bit Operations/Compare To Constant  Description=|  relop===  const=uint8(hex2dec('E7'))  OutDataTypeStr=uint8
      | shedingFuFa：只判断一个条件
      | 
      | 把输入与0xE7（十进制231）比较，使用关系“==”。成立输出1，不成立输出0；输出是判断标志，不是把输入缩放成该常数。
      | 
      | 这里识别一种指令编码。判断成立只说明指令匹配；父级还会结合有效帧、当前模式或其他允许条件决定是否更新。实际驱动要继续经过控制与板级输出，不能把1理解为硬件执行回执。
      settings: AttributesFormatString=shedingFuFa（设定副阀）
  shedingZhuFa : simulink/Logic and Bit Operations/Compare To Constant  Description=|  relop===  const=uint8(hex2dec('E6'))  OutDataTypeStr=uint8
      | shedingZhuFa：只判断一个条件
      | 
      | 把输入与0xE6（十进制230）比较，使用关系“==”。成立输出1，不成立输出0；输出是判断标志，不是把输入缩放成该常数。
      | 
      | 这里识别一种指令编码。判断成立只说明指令匹配；父级还会结合有效帧、当前模式或其他允许条件决定是否更新。实际驱动要继续经过控制与板级输出，不能把1理解为硬件执行回执。
      settings: AttributesFormatString=shedingZhuFa（设定主阀）
  shedingyingqi : simulink/Logic and Bit Operations/Compare To Constant  Description=|  relop===  const=uint8(hex2dec('E9'))  OutDataTypeStr=uint8
      | shedingyingqi：只判断一个条件
      | 
      | 把输入与0xE9（十进制233）比较，使用关系“==”。成立输出1，不成立输出0；输出是判断标志，不是把输入缩放成该常数。
      | 
      | 这里识别一种指令编码。判断成立只说明指令匹配；父级还会结合有效帧、当前模式或其他允许条件决定是否更新。实际驱动要继续经过控制与板级输出，不能把1理解为硬件执行回执。
      settings: AttributesFormatString=shedingyingqi（设定引气）
  shedingyoumen : simulink/Logic and Bit Operations/Compare To Constant  Description=|  relop===  const=uint8(hex2dec('E3'))  OutDataTypeStr=uint8
      | shedingyoumen：只判断一个条件
      | 
      | 把输入与0xE3（十进制227）比较，使用关系“==”。成立输出1，不成立输出0；输出是判断标志，不是把输入缩放成该常数。
      | 
      | 这里识别一种指令编码。判断成立只说明指令匹配；父级还会结合有效帧、当前模式或其他允许条件决定是否更新。实际驱动要继续经过控制与板级输出，不能把1理解为硬件执行回执。
      settings: AttributesFormatString=shedingyoumen（设定油门）
  shoudongjian : simulink/Logic and Bit Operations/Compare To Constant  Description=|  relop===  const=uint8(hex2dec('F2'))  OutDataTypeStr=uint8
      | shoudongjian：只判断一个条件
      | 
      | 把输入与0xF2（十进制242）比较，使用关系“==”。成立输出1，不成立输出0；输出是判断标志，不是把输入缩放成该常数。
      | 
      | 这里识别一种指令编码。判断成立只说明指令匹配；父级还会结合有效帧、当前模式或其他允许条件决定是否更新。实际驱动要继续经过控制与板级输出，不能把1理解为硬件执行回执。
      settings: AttributesFormatString=shoudongjian（手动减小）
  tingche : simulink/Logic and Bit Operations/Compare To Constant  Description=|  relop===  const=uint8(hex2dec('F0'))  OutDataTypeStr=uint8
      | tingche：只判断一个条件
      | 
      | 把输入与0xF0（十进制240）比较，使用关系“==”。成立输出1，不成立输出0；输出是判断标志，不是把输入缩放成该常数。
      | 
      | 这里识别一种指令编码。判断成立只说明指令匹配；父级还会结合有效帧、当前模式或其他允许条件决定是否更新。实际驱动要继续经过控制与板级输出，不能把1理解为硬件执行回执。
      settings: AttributesFormatString=tingche（停车）
  zijian : simulink/Logic and Bit Operations/Compare To Constant  Description=|  relop===  const=uint8(hex2dec('E1'))  OutDataTypeStr=uint8
      | zijian：只判断一个条件
      | 
      | 把输入与0xE1（十进制225）比较，使用关系“==”。成立输出1，不成立输出0；输出是判断标志，不是把输入缩放成该常数。
      | 
      | 这里识别一种指令编码。判断成立只说明指令匹配；父级还会结合有效帧、当前模式或其他允许条件决定是否更新。实际驱动要继续经过控制与板级输出，不能把1理解为硬件执行回执。
      settings: AttributesFormatString=zijian（自检）
  停车 : Gain  Gain=PG_Instr_Stop
  手动减 : Gain  Gain=PG_Instr_ManualrReduce
  手动加 : Gain  Gain=PG_Instr_ManualPlus
  指令更新 : Logic  AllPortsSameDT=off  OutDataTypeStr=boolean
  指令确认 : RelationalOperator  Operator===  OutDataTypeStr=boolean  InputSameDT=off
  檫除 : Gain  Gain=PG_Instr_Erase
  紧急停车 : Gain  Gain=PG_Instr_StopZero
  自检 : Gain  Gain=PG_Instr_SelfCheck
  装订和档位控制 : Subsystem  Description=|
      | 判断这帧是否在设置目标转速或选择档位
      | 
      | 两类编码被视为装订/档位指令：一类是命令值F3（十六进制）的直接装订；另一类是低8位为0D且取出的高8位档位号不超过12的档位命令。
      | 
      | 这里仅输出“属于这一类命令”的布尔标志，不计算具体转速。具体目标由Speed_Load_Cal继续从第5、6字节或档位表取出。例：直接装订F3可以进入目标解析，普通阀门命令不会因携带了数值就变成闭环目标。
  设定引气 : Gain  Gain=PG_Instr_BleedAirSet
  设定油路主阀 : Gain  Gain=PG_Instr_EValveSet
  设定油路副阀 : Gain  Gain=PG_Instr_EblastSet
  设定油门 : Gain  Gain=PG_Instr_OilSet
  设定点火器 : Gain  Gain=PG_Instr_FireWorkSet
  设定起动电机 : Gain  Gain=PG_Instr_MotorSet
  起动 : Gain  Gain=PG_Instr_Start
  闭环 : Gain  Gain=PG_Instr_CloseLoop
  S_Instr_XianShi : Outport
      settings: AttributesFormatString=S_Instr_XianShi（指令显示显示）
  S_Instr_Out : Outport  Port=2
      settings: AttributesFormatString=S_Instr_Out（指令输出）
  S_COMM_Data6 : Outport  Port=3
      settings: AttributesFormatString=S_COMM_Data6（通信数据6）
  wires:
  Switch1/1 -> Delay/1, S_Instr_XianShi/1
  S_Rx_suc/1 -> [Rx_suc]
  S_MyUsart2_Rxdata/1 -> [MyUsart2_Rxdata]
  [MyUsart2_Rxdata] -> COMM数组3位/1, COMM数组4位/1
  Switch/1 -> S_Instr_Out/1
  COMM数组4位/1 -> 指令确认/1
  指令确认/1 -> [Flag_Instr_suc]
  [Flag_Instr_suc] -> 指令更新/1
  [Rx_suc] -> 指令更新/2
  [MyUsart2_Rxdata] -> COMM数组6位/1
  COMM数组6位/1 -> S_COMM_Data6/1
  紧急停车/1 -> Add/15
  设定引气/1 -> Add/14
  设定起动电机/1 -> Add/13
  设定油路副阀/1 -> Add/12
  设定油路主阀/1 -> Add/11
  设定点火器/1 -> Add/10
  ECU重置/1 -> Add/9
  设定油门/1 -> Add/8
  自检/1 -> Add/7
  停车/1 -> Add/6
  手动减/1 -> Add/5
  手动加/1 -> Add/4
  闭环/1 -> Add/3
  起动/1 -> Add/2
  檫除/1 -> Add/1
  jinjitingche/1 -> 紧急停车/1
  shedingyingqi/1 -> 设定引气/1
  shedingDianJi/1 -> 设定起动电机/1
  shedingFuFa/1 -> 设定油路副阀/1
  shedingZhuFa/1 -> 设定油路主阀/1
  shedingDianHuoQi/1 -> 设定点火器/1
  装订和档位控制/1(S_Flagf_CLP) -> 闭环/1
  chongzhi/1 -> ECU重置/1
  shedingyoumen/1 -> 设定油门/1
  zijian/1 -> 自检/1
  tingche/1 -> 停车/1
  shoudongjian/1 -> 手动减/1
  ShouDongJia/1 -> 手动加/1
  qidong/1 -> 起动/1
  cachu/1 -> 檫除/1
  WuZhiLing/1 -> Switch/3
  Add/1 -> Switch/1
  指令更新/1 -> Switch/2
  Delay/1 -> Switch1/3
  COMM数组3位/1 -> qidong/1, shedingyingqi/1, jinjitingche/1, Switch1/1, shedingDianJi/1, shedingFuFa/1, shedingZhuFa/1, shedingDianHuoQi/1, chongzhi/1, shedingyoumen/1, zijian/1, tingche/1, shoudongjian/1, ShouDongJia/1, 装订和档位控制/1(S_COMM_Instr), cachu/1, 指令确认/2
  [Flag_Instr_suc] -> Switch1/2

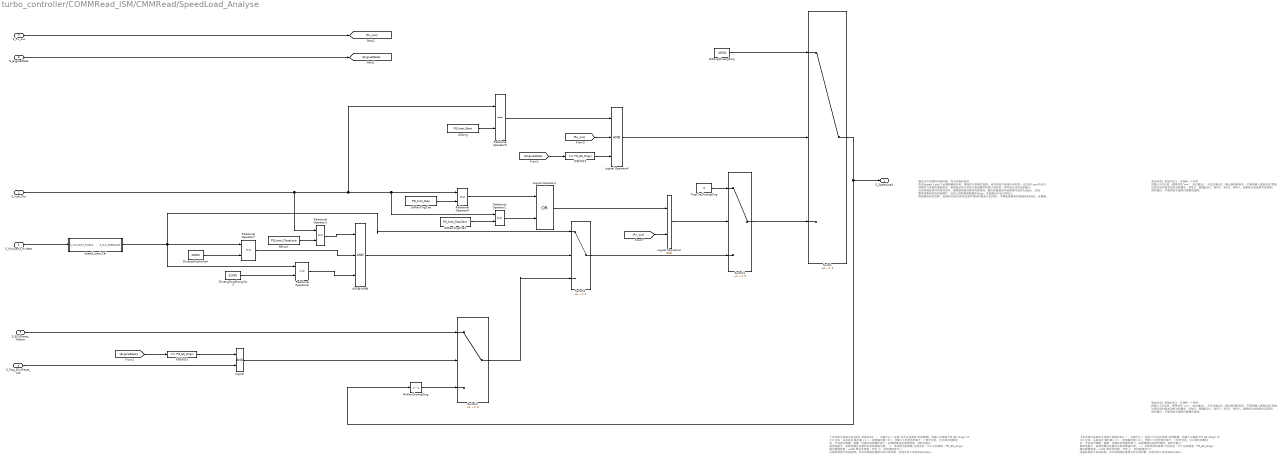
== system turbo_controller/COMMRead_ISM/CMMRead/SpeedLoad_Analyse ==
  note: 【本页库子系统中文说明】初始状态1
      | 一、它做什么？
      | 这是“过不过这条线”的判断器。将输入与阈值 PG_ES_Origin 作 == 比较，关系成立
      | 输出真（1），否则输出假（0）。例如>=包含恰好等于，>则不包含。它只给出判断标
      | 志，不会自行限幅、报警、切换状态或操作阀门；后续逻辑决定如何使用。名称可能只
      | 是用途提示，实际判据以这里的关系和阈值为准。
      | 二、本实例当前参数
      | 比较关系：==
      | 比较阈值：PG_ES_Origin
      | 输出数据类型：uint8
      | 零交叉检测：开启
      | 三、怎样继续学习？
      | 这是标准库子系统实例。中文说明放在使用它的父级页面，并同步存入本块Descriptio
      | n（模块说明）；官方库链接保留。先看本实例的输入来自哪里、输出交给谁，再结合
      | 以上参数理解作用。
  note: 【本页库子系统中文说明】初始状态2
      | 一、它做什么？
      | 这是“过不过这条线”的判断器。将输入与阈值 PG_ES_Origin 作 == 比较，关系成立
      | 输出真（1），否则输出假（0）。例如>=包含恰好等于，>则不包含。它只给出判断标
      | 志，不会自行限幅、报警、切换状态或操作阀门；后续逻辑决定如何使用。名称可能只
      | 是用途提示，实际判据以这里的关系和阈值为准。
      | 二、本实例当前参数
      | 比较关系：==
      | 比较阈值：PG_ES_Origin
      | 输出数据类型：uint8
      | 零交叉检测：开启
      | 三、怎样继续学习？
      | 这是标准库子系统实例。中文说明放在使用它的父级页面，并同步存入本块Descriptio
      | n（模块说明）；官方库链接保留。先看本实例的输入来自哪里、输出交给谁，再结合
      | 以上参数理解作用。
  note: 确定本次采用的目标转速，并记住有效目标
      |
      | 先由Speed_Load_Cal解码候选目标，再按命令和模式选择。闭环目标只有落在40000～61000 rpm的允许
      | 范围内才走相应更新路径；有效起动命令且处于初始模式时装订40000；停车命令走0目标路径。
      |
      | 当没有满足条件的新设定时，继续使用延迟保存的原目标。复位恢复路径可选择保存过的NcDem，但还
      | 要求恢复有效及初始模式；当前上层恢复使能固定false，这条路径不会正常投入。
      |
      | 例如原目标50000，新闭环目标55000且条件有效时更新为55000；不满足更新条件则继续50000。这里输
      | 出的是期望值，实际转速由传感器测得，CLM再对两者差值进行控制。
  note: 初始状态1
      | 初始状态1：只判断一个条件
      |
      | 把输入与0比较，使用关系“==”。成立输出1，不成立输出0；输出是判断标志，不是把输入缩放成该
      | 常数。
      |
      | 这里比较的是发动机当前模式：初始0、普通起动1、闭环2、手动3、停车4。结果供父级选择对应控制/
      | 保护路径，不能用命令编号代替模式编号。
  note: 初始状态2
      | 初始状态2：只判断一个条件
      |
      | 把输入与0比较，使用关系“==”。成立输出1，不成立输出0；输出是判断标志，不是把输入缩放成该
      | 常数。
      |
      | 这里比较的是发动机当前模式：初始0、普通起动1、闭环2、手动3、停车4。结果供父级选择对应控制/
      | 保护路径，不能用命令编号代替模式编号。
  S_Instr_Out : Inport
      settings: AttributesFormatString=S_Instr_Out（指令输出）
  S_Rx_suc : Inport  Port=2
      settings: AttributesFormatString=S_Rx_suc（接收数据成功或有效）
  S_MyUsart2_Rxdata : Inport  Port=3
      settings: AttributesFormatString=S_MyUsart2_Rxdata（四号串口指令缓冲区（沿用旧变量名））
  S_Flag_ECUReset_Use : Inport  Port=4
      settings: AttributesFormatString=S_Flag_ECUReset_Use（标志电子控制器复位使用）
  S_ECUReset_NcDem : Inport  Port=5
      settings: AttributesFormatString=S_ECUReset_NcDem（电子控制器复位目标转速）
  S_EngineState : Inport  Port=6
      settings: AttributesFormatString=S_EngineState（发动机状态）
  BiHuan : Constant  Value=PG_Instr_CloseLoop
      settings: AttributesFormatString=BiHuan（闭环）
  DiMianTingChe : Constant  Value=PG_Instr_Stop
      settings: AttributesFormatString=DiMianTingChe（地面停车）
  DiMianTingChe1 : Constant  Value=PG_Instr_StopZero
      settings: AttributesFormatString=DiMianTingChe1（地面停车1）
  "Logical " : Logic  AllPortsSameDT=off  OutDataTypeStr=boolean
      settings: AttributesFormatString=Logical （逻辑）
  Logical Operator1 : Logic  Operator=OR  AllPortsSameDT=off  OutDataTypeStr=boolean
      settings: AttributesFormatString=Logical Operator1（逻辑运算1）
  Logical Operator3 : Logic  AllPortsSameDT=off  OutDataTypeStr=boolean
      settings: AttributesFormatString=Logical Operator3（逻辑运算3）
  Logical Operator4 : Logic  Inputs=3  AllPortsSameDT=off  OutDataTypeStr=boolean
      settings: AttributesFormatString=Logical Operator4（逻辑运算4）
  MoRenZhuangDing : Delay  DelayLength=1  InitialCondition=0
      settings: AttributesFormatString=MoRenZhuangDing（默认装订参数）
  QiDong : Constant  Value=PG_Instr_Start
      settings: AttributesFormatString=QiDong（起动）
  QiDongZhuangDing : Constant  Value=40000  OutDataTypeStr=single
      settings: AttributesFormatString=QiDongZhuangDing（起动参数装订）
  Relational Operator{1..2,4..5} (4 alike) : RelationalOperator  Operator===  OutDataTypeStr=boolean  InputSameDT=off
      Relational Operator1 settings: AttributesFormatString=Relational Operator1（关系比较运算1）
      Relational Operator2 settings: AttributesFormatString=Relational Operator2（关系比较运算2）
      Relational Operator4 settings: AttributesFormatString=Relational Operator4（关系比较运算4）
      Relational Operator5 settings: AttributesFormatString=Relational Operator5（关系比较运算5）
  Relational Operator6 : RelationalOperator  Operator=<=  OutDataTypeStr=boolean  InputSameDT=off
      settings: AttributesFormatString=Relational Operator6（关系比较运算6）
  Relational Operator7 : RelationalOperator  OutDataTypeStr=boolean  InputSameDT=off
      settings: AttributesFormatString=Relational Operator7（关系比较运算7）
  Speed_Load_Cal : Subsystem  Description=|
      | 把直接装订或档位编码换算为目标转速
      | 
      | 直接装订：第3字节等于F3时，取第5、6字节，按高字节在前合成整数，再乘2。
      | 目标rpm = 2×(第5字节×256+第6字节)。
      | 例如高字节97、低字节168，合成25000，得到50000 rpm。
      | 
      | 档位路径：提取第3字节的高4位作为档位索引，按模型的一基索引从PF_Gear_Info表取目标；低位判定符合档位编码才采用，否则候选输出0。父级还会进行命令有效性和40000～61000范围选择。
      | 
      | 本模块只解码，不做转速闭环；无效候选0也不一定立刻把最终目标清零，父级可能保持旧目标。
      settings: AttributesFormatString=Speed_Load_Cal（档位及装订值换算目标转速）
  Switch{,1..3} (4 alike) : Switch  Criteria=u2 ~= 0  SaturateOnIntegerOverflow=off  InputSameDT=off
      settings: AttributesFormatString=Switch（开关选择）
  TingCheZhuangDing : Constant  Value=0  OutDataTypeStr=single
      settings: AttributesFormatString=TingCheZhuangDing（停车参数装订）
  ZhuangDingShangXian : Constant  Value=61000  OutDataTypeStr=uint32
      settings: AttributesFormatString=ZhuangDingShangXian（装订上限）
  ZhuangDingXiaXian : Constant  Value=40000  OutDataTypeStr=uint32
      settings: AttributesFormatString=ZhuangDingXiaXian（装订下限）
  初始状态1 : simulink/Logic and Bit Operations/Compare To Constant  Description=|  relop===  const=PG_ES_Origin  OutDataTypeStr=uint8
      | 初始状态1：只判断一个条件
      | 
      | 把输入与0比较，使用关系“==”。成立输出1，不成立输出0；输出是判断标志，不是把输入缩放成该常数。
      | 
      | 这里比较的是发动机当前模式：初始0、普通起动1、闭环2、手动3、停车4。结果供父级选择对应控制/保护路径，不能用命令编号代替模式编号。
  初始状态2 : simulink/Logic and Bit Operations/Compare To Constant  Description=|  relop===  const=PG_ES_Origin  OutDataTypeStr=uint8
      | 初始状态2：只判断一个条件
      | 
      | 把输入与0比较，使用关系“==”。成立输出1，不成立输出0；输出是判断标志，不是把输入缩放成该常数。
      | 
      | 这里比较的是发动机当前模式：初始0、普通起动1、闭环2、手动3、停车4。结果供父级选择对应控制/保护路径，不能用命令编号代替模式编号。
  "闭环指令判断 " : Logic  Inputs=3  AllPortsSameDT=off  OutDataTypeStr=boolean
  S_SpeedLoad : Outport
      settings: AttributesFormatString=S_SpeedLoad（装订转速）
  wires:
  S_MyUsart2_Rxdata/1 -> Speed_Load_Cal/1(S_MyUsart2_Rxdata)
  Relational Operator6/1 -> "闭环指令判断 "/3
  Relational Operator7/1 -> "闭环指令判断 "/2
  ZhuangDingShangXian/1 -> Relational Operator6/2
  ZhuangDingXiaXian/1 -> Relational Operator7/2
  Relational Operator1/1 -> "闭环指令判断 "/1
  BiHuan/1 -> Relational Operator1/2
  DiMianTingChe/1 -> Relational Operator4/2
  Switch/1 -> MoRenZhuangDing/1, S_SpeedLoad/1
  [Rx_suc] -> Logical Operator3/2
  [Rx_suc] -> Logical Operator4/2
  S_Rx_suc/1 -> [Rx_suc]
  S_Flag_ECUReset_Use/1 -> "Logical "/2
  初始状态2/1 -> Logical Operator4/3
  S_EngineState/1 -> [EngineState]
  [EngineState] -> 初始状态2/1
  初始状态1/1 -> "Logical "/1
  [EngineState] -> 初始状态1/1
  DiMianTingChe1/1 -> Relational Operator2/2
  Logical Operator1/1 -> Logical Operator3/1
  Relational Operator4/1 -> Logical Operator1/1
  Relational Operator2/1 -> Logical Operator1/2
  Relational Operator5/1 -> Logical Operator4/1
  S_Instr_Out/1 -> Relational Operator1/1, Relational Operator2/1, Relational Operator4/1, Relational Operator5/1
  QiDong/1 -> Relational Operator5/2
  Switch1/1 -> Switch/3
  QiDongZhuangDing/1 -> Switch/1
  Logical Operator4/1 -> Switch/2
  Switch2/1 -> Switch1/3
  TingCheZhuangDing/1 -> Switch1/1
  Logical Operator3/1 -> Switch1/2
  Switch3/1 -> Switch2/3
  Speed_Load_Cal/1(S_Out_SpeedLoad) -> Relational Operator6/1, Relational Operator7/1, Switch2/1
  "闭环指令判断 "/1 -> Switch2/2
  MoRenZhuangDing/1 -> Switch3/3
  S_ECUReset_NcDem/1 -> Switch3/1
  "Logical "/1 -> Switch3/2

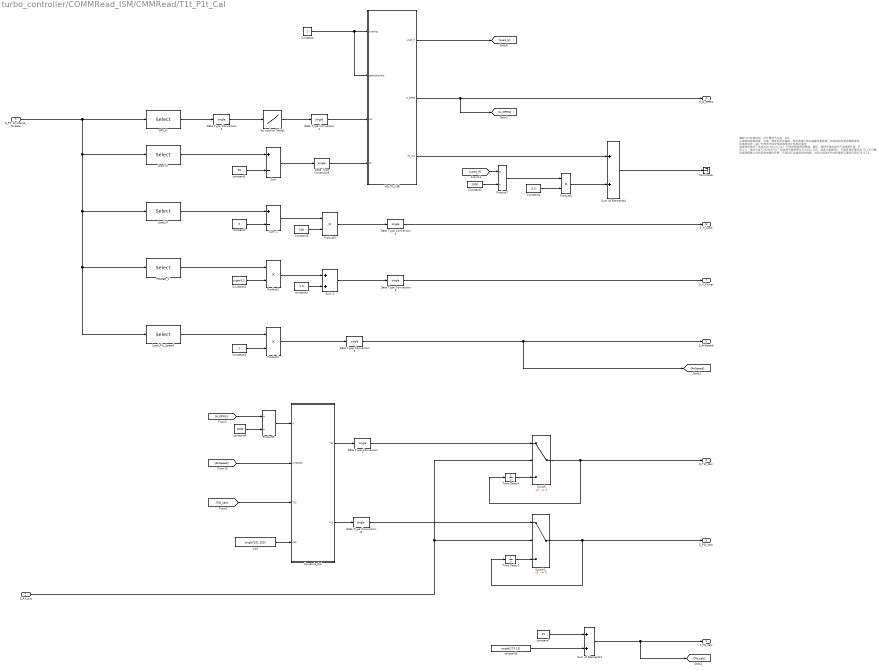
== system turbo_controller/COMMRead_ISM/CMMRead/T1t_P1t_Cal ==
  note: 解释飞行环境字段，并计算进气总温、总压
      |
      | 从通信帧提取高度、空速、温度及电压编码，按各通道比例与偏置恢复数值。有效接收时更新需要保持
      | 的高度信息；H0_T0图负责设定值和高度变化信息的保持。
      |
      | 高度由米换成千米后送Dynamic_Cal。它先按高度得到静温、静压，再把空速造成的气流减速升温、升
      | 压计入，输出总温T1t和总压P1t。标准海平面参考压力为101.325，温度计算要用K，不能直接把摄氏度
      | 代入平方根。
      |
      | 这里是根据上位机信息估算的环境，不是ADC总温电阻的换算。当前父级送ISM的转速修正温度仍采用28
      | 8.15 K常量，不能以为此处算出的总温已经接入所有下游控制。
  S_PF_MyUsart2_Rxdata : Inport
      settings: AttributesFormatString=S_PF_MyUsart2_Rxdata（本通道通用同步异步串行通信接口2接收数据）
  S_Rx_suc : Inport  Port=2
      settings: AttributesFormatString=S_Rx_suc（接收数据成功或有效）
  Constant : Constant  OutDataTypeStr=boolean
      settings: AttributesFormatString=Constant（常量）
  Constant1 : Constant  Value=6.5  OutDataTypeStr=single
      settings: AttributesFormatString=Constant1（常量1）
  Constant2 : Constant  Value=1000  OutDataTypeStr=single
      settings: AttributesFormatString=Constant2（常量2）
  Constant3 : Constant  Value=2  OutDataTypeStr=single
      settings: AttributesFormatString=Constant3（常量3）
  Constant4 : Constant  Value=single(0.2)  OutDataTypeStr=single
      settings: AttributesFormatString=Constant4（常量4）
  Constant5 : Constant  Value=100  OutDataTypeStr=single
      settings: AttributesFormatString=Constant5（常量5）
  Data Type Conersion6 : DataTypeConversion  OutDataTypeStr=single  SaturateOnIntegerOverflow=off  RndMeth=Floor
      settings: AttributesFormatString=Data Type Conersion6（数据类型转换6）
  Data Type Conversion{1..5,7..8} (7 alike) : DataTypeConversion  OutDataTypeStr=single  SaturateOnIntegerOverflow=off  RndMeth=Floor
      Data Type Conversion1 settings: AttributesFormatString=Data Type Conversion1（数据类型转换1）
      Data Type Conversion2 settings: AttributesFormatString=Data Type Conversion2（数据类型转换2）
      Data Type Conversion3 settings: AttributesFormatString=Data Type Conversion3（数据类型转换3）
      Data Type Conversion4 settings: AttributesFormatString=Data Type Conversion4（数据类型转换4）
      Data Type Conversion5 settings: AttributesFormatString=Data Type Conversion5（数据类型转换5）
      Data Type Conversion7 settings: AttributesFormatString=Data Type Conversion7（数据类型转换7）
      Data Type Conversion8 settings: AttributesFormatString=Data Type Conversion8（数据类型转换8）
  Dynamic_Cal : Subsystem  Description=|
      | 由高度和空速分两步估算进气总温、总压
      | 
      | 第一步P1H_T1H：输入高度H（km）、参考温度T10（K）、参考压力p10，计算该高度的静温T1H和静压P1H，描述未被进气道减速前的外界空气。
      | 
      | 第二步dynamic：把T1H、P1H与空速AirSpeed（m/s）一起计算，得到气流理想减速到零速度时的总温T1t、总压P1t。速度越高，动能转化引起的总温与总压增加越明显。
      | 
      | 例如H=0、空速=0时，总温等于参考温度，总压等于参考压力。空速不为0时，不能只按高度算静压后就把它称为总压。公式及适用假设分别写在下面两个子系统内部。
      settings: AttributesFormatString=Dynamic_Cal（动态计算）
  GPS_H : Selector  IndexMode=Zero-based  InputPortWidth=50  IndexOptions=Index vector (dialog)  Indices=[6]  OutputSizes=1
      settings: AttributesFormatString=GPS_H（导航高度）
  H0_T0_计算 : Stateflow chart  Description=|  TreatAsAtomicUnit=on
      | 保持环境设定，并按更新条件刷新高度信息
      | 
      | sheding条件满足时，把输入H0保存到Load_H，把输入T0保存到T0_out；gaodubianhua条件满足时，把H0保存到H_GPRS。条件不满足时不重新赋值，输出继续保留上次结果。
      | 
      | 当前父级把这两个条件都接到接收更新相关信号，因此更新时机取决于通信帧。两个高度输出虽然都取自H0，供下游使用的用途不同；不能把它们的名称理解为本图重新计算了两套GPS位置。
      | 
      | 本处不执行大气公式，温度转K、高度转km以及总温总压计算在外层完成。
      settings: AttributesFormatString=H0_T0_计算（初始高度环境温度计算）
  Kp Lookup Table1 : Lookup_n-D  NumberOfTableDimensions=1  BreakpointsForDimension1=[0 205]  Table=[-500 20000]  ExtrapMethod=Clip  UseLastTableValue=on  InternalRulePriority=Speed  RndMeth=Simplest
      settings: AttributesFormatString=Kp Lookup Table1（比例系数查找表1）
  LoadT0 : Selector  IndexMode=Zero-based  InputPortWidth=50  IndexOptions=Index vector (dialog)  Indices=[7]  OutputSizes=1
      settings: AttributesFormatString=LoadT0（负载或装订值温度、时间或真分支输入0）
  Load_Fly_Speed : Selector  IndexMode=Zero-based  InputPortWidth=50  IndexOptions=Index vector (dialog)  Indices=[9]  OutputSizes=1
      settings: AttributesFormatString=Load_Fly_Speed（负载或装订值飞行速度或转速）
  Load_H : Selector  IndexMode=Zero-based  InputPortWidth=50  IndexOptions=Index vector (dialog)  Indices=[11]  OutputSizes=1
      settings: AttributesFormatString=Load_H（装订高度）
  POWER_V : Selector  IndexMode=Zero-based  InputPortWidth=50  IndexOptions=Index vector (dialog)  Indices=[10]  OutputSizes=1
      settings: AttributesFormatString=POWER_V（电源电压或控制量变量）
  Product{1..3,6} (4 alike) : Product  Inputs=**
      Product1 settings: AttributesFormatString=Product1（乘法1）
      Product2 settings: AttributesFormatString=Product2（乘法2）
      Product3 settings: AttributesFormatString=Product3（乘法3）
      Product6 settings: AttributesFormatString=Product6（乘法6）
  Product5 : Product  Inputs=*/
      settings: AttributesFormatString=Product5（乘法5）
  Product7 : Product  Inputs=*/
      settings: AttributesFormatString=Product7（乘法7）
  "Sum " : Sum  Inputs=+-
      settings: AttributesFormatString=Sum （加法求和）
  Sum 1 : Sum  Inputs=+-
      settings: AttributesFormatString=Sum 1（加法求和1）
  Sum 2 : Sum
      settings: AttributesFormatString=Sum 2（加法求和2）
  Sum of Elements1 : Sum
      settings: AttributesFormatString=Sum of Elements1（加法求和的元素1）
  Sum of Elements4 : Sum
      settings: AttributesFormatString=Sum of Elements4（加法求和的元素4）
  Switch : Switch  Criteria=u2 ~= 0  SaturateOnIntegerOverflow=off  InputSameDT=off
      settings: AttributesFormatString=Switch（开关选择）
  Switch1 : Switch  Criteria=u2 ~= 0  SaturateOnIntegerOverflow=off  InputSameDT=off
      settings: AttributesFormatString=Switch（开关选择）
  Terminator : Terminator
      settings: AttributesFormatString=Terminator（终止未使用信号）
  Time Delay1 : UnitDelay  InitialCondition=single(288.15)  SampleTime=-1  HasFrameUpgradeWarning=on
      settings: AttributesFormatString=Time Delay1（时间延迟1）
  Time Delay4 : UnitDelay  InitialCondition=single(288.15)  SampleTime=-1  HasFrameUpgradeWarning=on
      settings: AttributesFormatString=Time Delay4（时间延迟4）
  constant1 : Constant  Value=50  OutDataTypeStr=single  SampleTime=-1
      settings: AttributesFormatString=constant1（常量1）
  constant2 : Constant  Value=5  OutDataTypeStr=single  SampleTime=-1
      settings: AttributesFormatString=constant2（常量2）
  constant3 : Constant  Value=single(273.15)  OutDataTypeStr=single  SampleTime=-1
      settings: AttributesFormatString=constant3（常量3）
  constant4 : Constant  Value=1000  OutDataTypeStr=single  SampleTime=-1
      settings: AttributesFormatString=constant4（常量4）
  constant5 : Constant  Value=1.5  OutDataTypeStr=single  SampleTime=-1
      settings: AttributesFormatString=constant5（常量5）
  constant7 : Constant  Value=15  OutDataTypeStr=single  SampleTime=-1
      settings: AttributesFormatString=constant7（常量7）
  p10 : Constant  Value=single(101.325)  OutDataTypeStr=single  SampleTime=-1
      settings: AttributesFormatString=p10（压力或比例变量10）
  S_T0_calc : Outport
      settings: AttributesFormatString=S_T0_calc（环境温度计算）
  S_T1t_calc : Outport  Port=2
      settings: AttributesFormatString=S_T1t_calc（入口总温计算）
  S_P1t_calc : Outport  Port=3
      settings: AttributesFormatString=S_P1t_calc（入口总压计算）
  S_H_GPRS : Outport  Port=4
      settings: AttributesFormatString=S_H_GPRS（导航高度）
  S_AirSpeed : Outport  Port=5
      settings: AttributesFormatString=S_AirSpeed（空速）
  S_H_Load : Outport  Port=6
      settings: AttributesFormatString=S_H_Load（装订高度）
  S_V_Power : Outport  Port=7
      settings: AttributesFormatString=S_V_Power（电压或控制量变量电源）
  wires:
  p10/1 -> Dynamic_Cal/4(p10)
  Dynamic_Cal/1(T1t) -> Data Type Conversion7/1
  [AirSpeed] -> Dynamic_Cal/2(AirSpeed)
  constant3/1 -> Sum of Elements1/2
  S_PF_MyUsart2_Rxdata/1 -> Load_Fly_Speed/1, POWER_V/1, Load_H/1, LoadT0/1, GPS_H/1
  Sum of Elements1/1 -> [T0t_calc], S_T0_calc/1
  Load_Fly_Speed/1 -> Product1/1
  Data Type Conversion5/1 -> [AirSpeed], S_AirSpeed/1
  [H_GPRS] -> Product5/1
  Product5/1 -> Dynamic_Cal/1(H)
  constant4/1 -> Product5/2
  Constant1/1 -> Product6/2
  Product6/1 -> Sum of Elements4/2
  Product7/1 -> Product6/1
  [Load_H] -> Product7/1
  Constant2/1 -> Product7/2
  Switch/1 -> S_T1t_calc/1, Time Delay4/1
  Switch1/1 -> Time Delay1/1, S_P1t_calc/1
  Dynamic_Cal/2(P1t) -> Data Type Conversion8/1
  H0_T0_计算/1(Load_H) -> [Load_H]
  Constant3/1 -> Product1/2
  Product1/1 -> Data Type Conversion5/1
  GPS_H/1 -> Data Type Conversion2/1
  Kp Lookup Table1/1 -> Data Type Conversion1/1
  Constant/1 -> H0_T0_计算/2(gaodubianhua), H0_T0_计算/1(sheding)
  H0_T0_计算/2(H_GPRS) -> [H_GPRS], S_H_GPRS/1
  H0_T0_计算/3(T0_out) -> Sum of Elements4/1
  Data Type Conversion1/1 -> H0_T0_计算/3(H0)
  Data Type Conversion2/1 -> Kp Lookup Table1/1
  Load_H/1 -> Sum 1/1
  Data Type Conversion3/1 -> S_V_Power/1
  Data Type Conversion4/1 -> S_H_Load/1
  Product3/1 -> Data Type Conversion4/1
  Constant4/1 -> Product2/2
  Product2/1 -> Sum 2/1
  POWER_V/1 -> Product2/1
  constant2/1 -> Sum 1/2
  Constant5/1 -> Product3/2
  Sum 1/1 -> Product3/1
  constant5/1 -> Sum 2/2
  Sum 2/1 -> Data Type Conversion3/1
  Data Type Conersion6/1 -> H0_T0_计算/4(T0)
  constant1/1 -> "Sum "/2
  "Sum "/1 -> Data Type Conersion6/1
  LoadT0/1 -> "Sum "/1
  [T0t_calc] -> Dynamic_Cal/3(T10)
  constant7/1 -> Sum of Elements1/1
  Sum of Elements4/1 -> Terminator/1
  Time Delay4/1 -> Switch/3
  Data Type Conversion7/1 -> Switch/1
  Time Delay1/1 -> Switch1/3
  Data Type Conversion8/1 -> Switch1/1
  S_Rx_suc/1 -> Switch/2, Switch1/2
